simulink model "BESS_GFM_PV_GFL_Stage1_R1_3_PV_POWER_READABLE"  (R2026a)
settings: Solver=ode23t  StopTime=0.9  MaxStep=1e-5
InitFcn:
  | run(fullfile(fileparts(get_param(bdroot,'FileName')),'..','scripts','init_bess_pv_stage1_r1.m'));
undefined symbols (not defined in the file): Control, G, S1, S21
libraries: ee_lib x19, nesl_utility x16, fl_lib x9, simulink x3, sl_discontinuities x1
settings Model: Creator=fakebob2004  LastModifiedBy=fakebob2004
settings SimscapeCC: SimscapeLogType=none

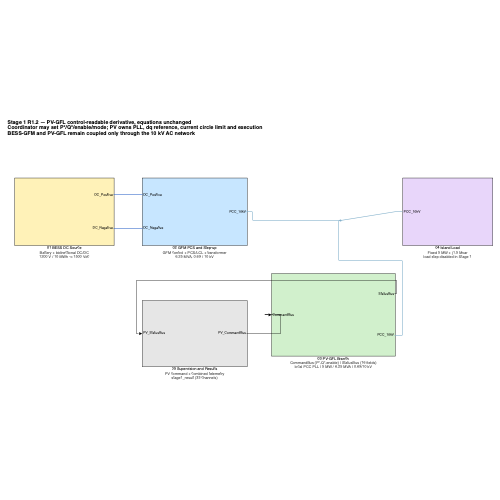
[thumbnail: Simulink's stored preview of the top-level diagram]
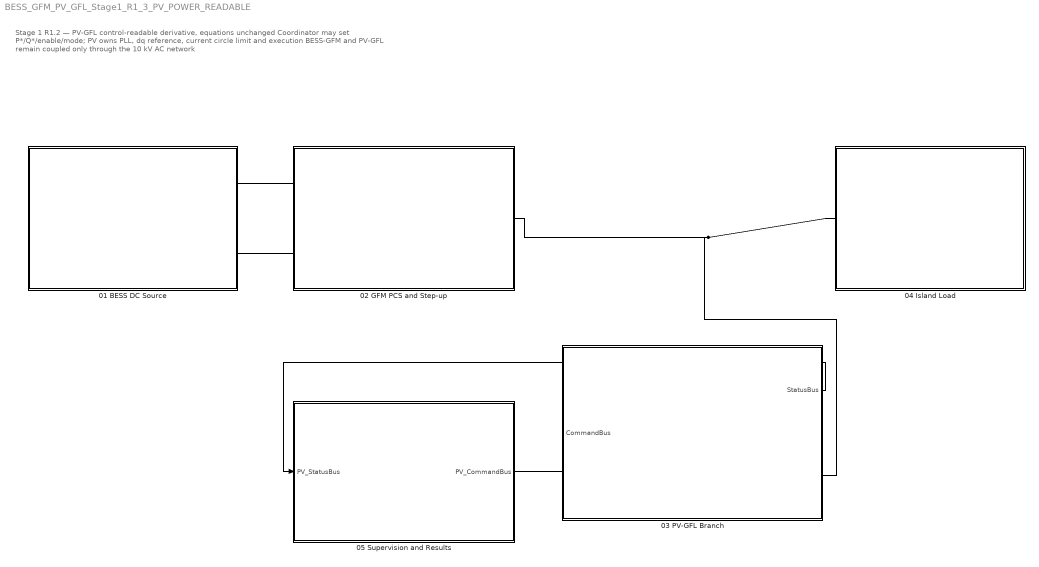
== system BESS_GFM_PV_GFL_Stage1_R1_3_PV_POWER_READABLE ==
  note: Stage 1 R1.2 — PV-GFL control-readable derivative, equations unchanged
      | Coordinator may set P*/Q*/enable/mode; PV owns PLL, dq reference, current circle limit and execution
      | BESS-GFM and PV-GFL remain coupled only through the 10 kV AC network
  01 BESS DC Source : Subsystem
      settings: AttributesFormatString=Battery + bidirectional DC/DC\n1200 V / 10 MWh -> 1500 Vdc
  02 GFM PCS and Step-up : Subsystem
      settings: AttributesFormatString=GFM control + PCS/LCL + transformer\n6.25 MVA, 0.69 / 10 kV
  03 PV-GFL Branch : Subsystem
      settings: AttributesFormatString=|
      | CommandBus {P*,Q*,enable} | StatusBus {16 fields}
      | local PCC PLL | 5 MW / 6.25 MVA | 0.69/10 kV
  04 Island Load : Subsystem
      settings: AttributesFormatString=Fixed 5 MW + j1.5 Mvar\nload step disabled in Stage 1
  05 Supervision and Results : Subsystem
      settings: AttributesFormatString=PV command + combined telemetry\nstage1_result (33 channels)
  wires:
  05 Supervision and Results/1(PV_CommandBus) -> 03 PV-GFL Branch/1(CommandBus)
  03 PV-GFL Branch/1(StatusBus) -> 05 Supervision and Results/1(PV_StatusBus)
  connections:
  01 BESS DC Source/RConn1 -- 02 GFM PCS and Step-up/LConn1
  01 BESS DC Source/RConn2 -- 02 GFM PCS and Step-up/LConn2
  04 Island Load/LConn1 -- 02 GFM PCS and Step-up/RConn1 -- 03 PV-GFL Branch/RConn1

== system BESS_GFM_PV_GFL_Stage1_R1_3_PV_POWER_READABLE/01 BESS DC Source ==
  01 Battery and DC Link : Subsystem
      settings: AttributesFormatString=1200 V / 10 MWh\n1500 V DC link
  02 Bidirectional DC-DC Control : Subsystem
      settings: AttributesFormatString=Vdc PI: 10 Hz\nIbat PI: 300 Hz
  DC_Positive : PMIOPort  Side=Right  ConnectionType=Connection: foundation.electrical.electrical
  DC_Negative : PMIOPort  Port=2  Side=Right  ConnectionType=Connection: foundation.electrical.electrical
  connections:
  02 Bidirectional DC-DC Control/RConn1 -- 01 Battery and DC Link/LConn2
  01 Battery and DC Link/RConn2 -- DC_Negative/RConn1
  DC_Positive/RConn1 -- 01 Battery and DC Link/LConn1

== system BESS_GFM_PV_GFL_Stage1_R1_3_PV_POWER_READABLE/02 GFM PCS and Step-up ==
  03 GFM Control and Limits : Subsystem
      settings: AttributesFormatString=P-f / Q-V / Virtual Z\nAC limit: 1.20 pu
  04 PCS Filter and Transformer : Subsystem
      settings: AttributesFormatString=6.25 MVA PCS + LCL\n0.69 / 10 kV transformer
  DC_Positive : PMIOPort  Side=Left  ConnectionType=Connection: foundation.electrical.electrical
  DC_Negative : PMIOPort  Port=2  Side=Left  ConnectionType=Connection: foundation.electrical.electrical
  PCC_10kV : PMIOPort  Port=3  Side=Right  ConnectionType=Connection: foundation.electrical.three_phase
  connections:
  04 PCS Filter and Transformer/RConn3 -- DC_Negative/RConn1
  04 PCS Filter and Transformer/RConn2 -- PCC_10kV/RConn1
  04 PCS Filter and Transformer/RConn1 -- DC_Positive/RConn1
  03 GFM Control and Limits/RConn1 -- 04 PCS Filter and Transformer/LConn1

== system BESS_GFM_PV_GFL_Stage1_R1_3_PV_POWER_READABLE/03 PV-GFL Branch ==
  CommandBus : Inport
  01 GFL PCS : Subsystem
      settings: AttributesFormatString=|
      | local fast control + average PCS/filter
      | no shared theta, PLL or DC link
  02 Step-up and PCC : Subsystem
      settings: AttributesFormatString=|
      | POWER: 690 V -> 0.69/10 kV -> PCC sensor -> 10 kV
      | MEASUREMENT: local V/I/P/Q -> PCC MeasurementBus
  scope_R21_CurrentCommandBus : GotoTagVisibility  GotoTag=R21_CurrentCommandBus
  scope_R21_PCCMeasurementBus : GotoTagVisibility  GotoTag=R21_PCCMeasurementBus
  scope_R21_PrimaryMeasurementBus : GotoTagVisibility  GotoTag=R21_PrimaryMeasurementBus
  PCC_10kV : PMIOPort  Side=Right  ConnectionType=Connection: foundation.electrical.three_phase
  StatusBus : Outport
  wires:
  01 GFL PCS/1(StatusBus) -> StatusBus/1
  CommandBus/1 -> 01 GFL PCS/1(CommandBus)
  connections:
  01 GFL PCS/RConn1 -- 02 Step-up and PCC/LConn1
  02 Step-up and PCC/RConn1 -- PCC_10kV/RConn1

== system BESS_GFM_PV_GFL_Stage1_R1_3_PV_POWER_READABLE/04 Island Load ==
  Adjusted_Island_Load : ee_lib/Passive/Constant Power Load (Three-Phase)  port_option=ee.enum.threePhasePort.composite  FRated=G.f0_Hz Hz  active_power=G.load.base_P_W W  reactive_power=G.load.base_Q_var V*A  Vline_rms_min=0.70*G.ac.Vll_high_V V  tau=0.01 s  Vline_rms_ini=G.ac.Vll_high_V V  Vang_ini=0 deg  gmin=1e-6 S
  Load_Step_Command : Step  Time=G.load.step_time_s  InitialValue=1  FinalValue=0  SampleTime=0
  Load_Step_to_PS : nesl_utility/Simulink-PS Converter  PhysicalDomain=network_engine_domain  SubClassName=ps_input  LeftPortType=input  RightPortType=output  PseudoPeriodic=off  Frequencies=[]  NoiseDistribution=none  NoiseParameters=[]  Unit=V  AffineConversion=off  FilteringAndDerivatives=zero  SimscapeFilterOrder=1  InputFilterTimeConstant=0.001  UdotUserProvided=0
  One_MW_Step_Load : ee_lib/Passive/Constant Power Load (Three-Phase)  port_option=ee.enum.threePhasePort.composite  FRated=G.f0_Hz Hz  active_power=0 W  reactive_power=0 V*A  Vline_rms_min=0.70*G.ac.Vll_high_V V  tau=0.01 s  Vline_rms_ini=G.ac.Vll_high_V V  Vang_ini=0 deg  gmin=1e-6 S
  Step_Load_Breaker : ee_lib/Switches & Breakers/Circuit Breaker (Three-Phase)  port_option=ee.enum.threePhasePort.composite  control_port_option=ee.enum.controlport.ps  R_closed=0.001 Ohm  G_open=1e-6 1/Ohm  threshold=0.5 V  breaker_behavior=ee.enum.switches.breakerBehavior.zeroCrossingEnable  i_th=1e-8 A
  PCC_10kV : PMIOPort  Side=Left  ConnectionType=Connection: foundation.electrical.three_phase
  tag scope: R8_05_Island_Load_Scenario_p1_signal=global
  wires:
  Load_Step_Command/1 -> Load_Step_to_PS/1, [R8_05_Island_Load_Scenario_p1_signal]  "step_breaker_cmd"
  connections:
  Step_Load_Breaker/RConn1 -- One_MW_Step_Load/LConn1
  PCC_10kV/RConn1 -- Adjusted_Island_Load/LConn1 -- Step_Load_Breaker/LConn2
  Load_Step_to_PS/RConn1 -- Step_Load_Breaker/LConn1

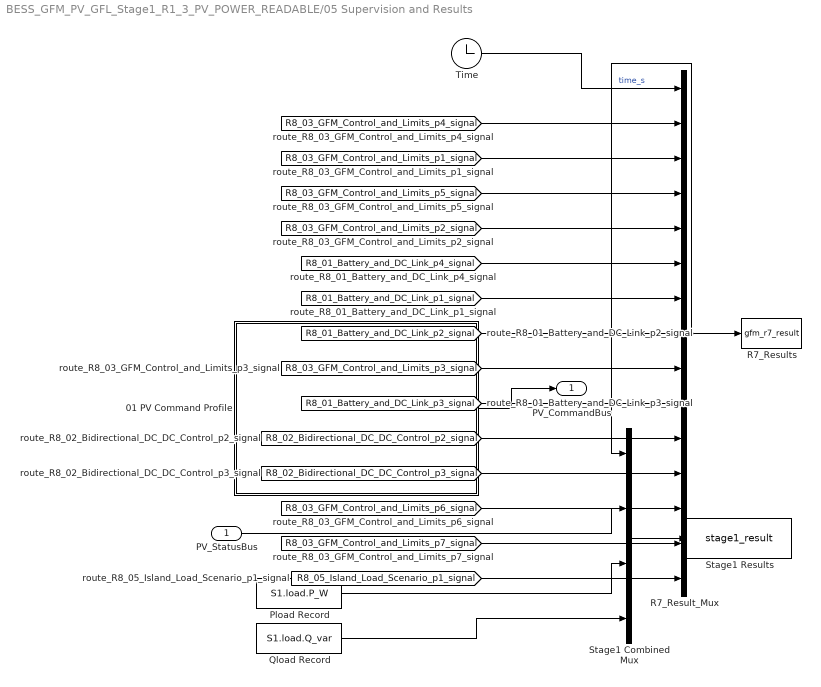
== system BESS_GFM_PV_GFL_Stage1_R1_3_PV_POWER_READABLE/05 Supervision and Results ==
  PV_StatusBus : Inport
  01 PV Command Profile : Subsystem
      settings: AttributesFormatString=|
      | CommandBus = [P*, Q*, enable]
      | commissioning scenario only
  Pload Record : Constant  Value=S1.load.P_W
  Qload Record : Constant  Value=S1.load.Q_var
  R7_Result_Mux : Mux  Inputs=15
  R7_Results : ToWorkspace  VariableName=gfm_r7_result  SampleTime=-1
  Stage1 Combined Mux : Mux
  Stage1 Results : ToWorkspace  VariableName=stage1_result  SampleTime=-1
  Time : Clock
  PV_CommandBus : Outport
  wires:
  [R8_05_Island_Load_Scenario_p1_signal] -> R7_Result_Mux/15
  [R8_03_GFM_Control_and_Limits_p7_signal] -> R7_Result_Mux/14
  R7_Result_Mux/1 -> R7_Results/1, Stage1 Combined Mux/1
  [R8_03_GFM_Control_and_Limits_p6_signal] -> R7_Result_Mux/13
  [R8_02_Bidirectional_DC_DC_Control_p3_signal] -> R7_Result_Mux/12
  [R8_02_Bidirectional_DC_DC_Control_p2_signal] -> R7_Result_Mux/11
  [R8_01_Battery_and_DC_Link_p3_signal] -> R7_Result_Mux/10
  [R8_03_GFM_Control_and_Limits_p3_signal] -> R7_Result_Mux/9
  [R8_01_Battery_and_DC_Link_p2_signal] -> R7_Result_Mux/8
  [R8_01_Battery_and_DC_Link_p1_signal] -> R7_Result_Mux/7
  [R8_01_Battery_and_DC_Link_p4_signal] -> R7_Result_Mux/6
  [R8_03_GFM_Control_and_Limits_p2_signal] -> R7_Result_Mux/5
  Time/1 -> R7_Result_Mux/1  "time_s"
  [R8_03_GFM_Control_and_Limits_p5_signal] -> R7_Result_Mux/4
  [R8_03_GFM_Control_and_Limits_p1_signal] -> R7_Result_Mux/3
  [R8_03_GFM_Control_and_Limits_p4_signal] -> R7_Result_Mux/2
  01 PV Command Profile/1(CommandBus Out) -> PV_CommandBus/1
  PV_StatusBus/1 -> Stage1 Combined Mux/2
  Pload Record/1 -> Stage1 Combined Mux/3
  Qload Record/1 -> Stage1 Combined Mux/4
  Stage1 Combined Mux/1 -> Stage1 Results/1

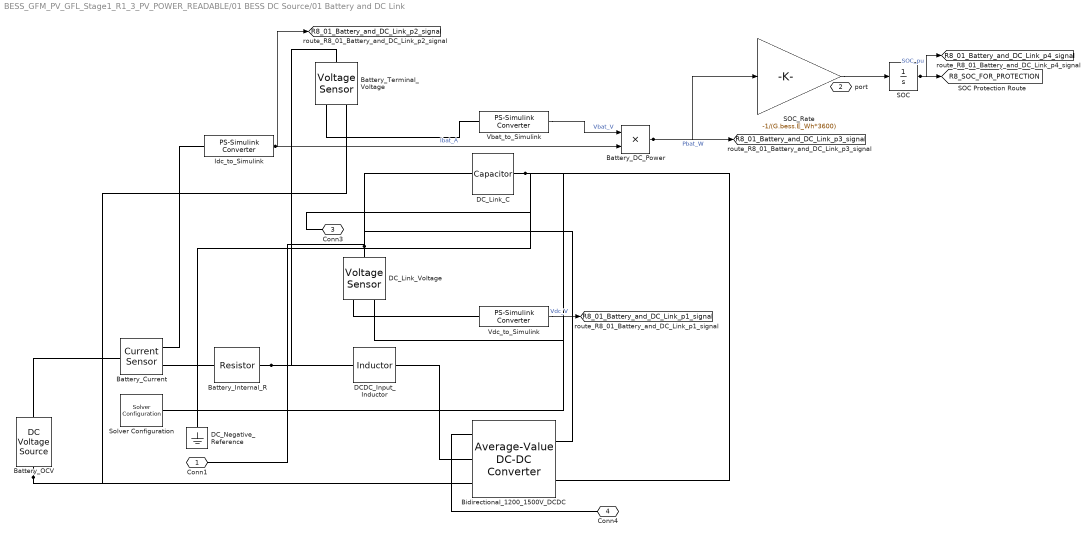
== system BESS_GFM_PV_GFL_Stage1_R1_3_PV_POWER_READABLE/01 BESS DC Source/01 Battery and DC Link ==
  Battery_Current : fl_lib/Electrical/Electrical Sensors/Current Sensor
  Battery_DC_Power : Product
  Battery_Internal_R : fl_lib/Electrical/Electrical Elements/Resistor  R=G.dc.Rbattery_ohm Ohm  i_specify=off  i_priority=None  i=0 A  i_nominal_specify=off  i_nominal_value=1  i_nominal_unit=A  v_specify=off  v_priority=None  v=0 V  v_nominal_specify=off  v_nominal_value=1  v_nominal_unit=V
  Battery_OCV : fl_lib/Electrical/Electrical Sources/DC Voltage Source  v0=G.dc.Vbattery_V V
  Battery_Terminal_Voltage : fl_lib/Electrical/Electrical Sensors/Voltage Sensor
  Bidirectional_1200_1500V_DCDC : ee_lib/Semiconductors & Converters/Converters/Average-Value DC-DC Converter  implementation_option=ee.enum.converters.implementation.behavioral  converter_type=ee.enum.converters.dcdctype.buckboost  control_option=ee.enum.converters.controlinput.dutycycle  efficiency_option=ee.enum.converters.efficiency.constant  efficiency_fixed=G.dc.dcdc_efficiency_pct  i_vec=[0, 2, 5] A  efficiency_vec=[90, 95, 98]  Lf=1e-6 H  Rl=0 Ohm  Cf=1e-7 F  Rc=1e-6 Ohm  iL_specify=off  iL_priority=High  iL=0 A  iL_nominal_specify=off  iL_nominal_value=1  iL_nominal_unit=A  vc_specify=off  vc_priority=High  vc=0 V  vc_nominal_specify=off  vc_nominal_value=1  vc_nominal_unit=V
  DCDC_Input_Inductor : fl_lib/Electrical/Electrical Elements/Inductor  l=G.dcdc.L_H H  r=0 Ohm  g=1e-9 1/Ohm  i_specify=on  i_priority=None  i=G.dcdc.Iref_initial_A A  i_nominal_specify=off  i_nominal_value=1  i_nominal_unit=A  v_specify=off  v_priority=None  v=0 V  v_nominal_specify=off  v_nominal_value=1  v_nominal_unit=V  i_L_specify=off  i_L_priority=High  i_L=0 A  i_L_nominal_specify=off  i_L_nominal_value=1  i_L_nominal_unit=A
  DC_Link_C : fl_lib/Electrical/Electrical Elements/Capacitor  c=G.dc.Cdc_F F  r=1e-6 Ohm  g=0 1/Ohm  i_specify=off  i_priority=None  i=0 A  i_nominal_specify=off  i_nominal_value=1  i_nominal_unit=A  v_specify=off  v_priority=None  v=0 V  v_nominal_specify=off  v_nominal_value=1  v_nominal_unit=V  vc_specify=on  vc_priority=High  vc=G.dc.Vdc_ref_V V  vc_nominal_specify=off  vc_nominal_value=1  vc_nominal_unit=V
  DC_Link_Voltage : fl_lib/Electrical/Electrical Sensors/Voltage Sensor
  DC_Negative_Reference : fl_lib/Electrical/Electrical Elements/Electrical Reference
  Idc_to_Simulink : nesl_utility/PS-Simulink Converter  PhysicalDomain=network_engine_domain  SubClassName=ps_output  LeftPortType=input  RightPortType=output  PseudoPeriodic=off  Frequencies=[]  VectorFormat=inherit  Unit=A  AffineConversion=off
  SOC : Integrator  InitialCondition=G.bess.SOC0  LimitOutput=on  UpperSaturationLimit=G.bess.SOC_max  LowerSaturationLimit=G.bess.SOC_min
  SOC_Rate : Gain  Gain=-1/(G.bess.E_Wh*3600)
  Solver Configuration : nesl_utility/Solver Configuration  PhysicalDomain=network_engine_domain  SubClassName=solver  LeftPortType=input  RightPortType=generic  Tones=[]  Harmonics=[]  SimulateNoise=off  Profile=off  UseLocalSampling=off  EnableSwitchedLinearOptims=on  FrequencyDomain=off  UseCCode=off  RelTol=0.001  AbsTol=0.001  MinStep=1e-09  ToWorkspace=off  RevertToSquareIcSolve=off  NumHomotopyIterations=100  PhasorMode=off  PhasorModeNumHarmonics=1  ConsistencySolver=NEWTON_XTOL_AFTER_FTOL  CanonicalOrdering=CANONICAL  OptimizeIntermediates=OPTIMIZED  IndexReductionMethod=DerivativeReplacement  DoDC=off  ResidualTolerance=1e-09  ConsistencyTolSource=GLOBAL  ConsistencyAbsTol=0.001  ConsistencyRelTol=0.001  ConsistencyTolFactor=0.001  UseLocalSolver=off  LocalSolverChoice=NE_BACKWARD_EULER_ADVANCER  ResolveIndetEquations=on  FunctionEvalNumThread=1  LocalSolverSampleTime=0.001  DoFixedCost=off  MaxNonlinIter=3  MaxModeIter=2  ComputeImpulses=off  ImpulseIterations=2  LinearAlgebra=auto  LinearAlgebraNumThread=0  EquationFormulation=NE_TIME_EF  DelaysMemoryBudget=1024  AutomaticFiltering=on  FilteringTimeConstant=0.001  PartitionStorageMethod=AS_NEEDED  PartitionMemoryBudget=1024  PartitionMethod=ROBUST  MultibodyUseLocalSolver=off  MultibodyLocalSolverChoice=ODE1  MultibodyLocalSolverSampleTime=0.001
  Vbat_to_Simulink : nesl_utility/PS-Simulink Converter  PhysicalDomain=network_engine_domain  SubClassName=ps_output  LeftPortType=input  RightPortType=output  PseudoPeriodic=off  Frequencies=[]  VectorFormat=inherit  Unit=V  AffineConversion=off
  Vdc_to_Simulink : nesl_utility/PS-Simulink Converter  PhysicalDomain=network_engine_domain  SubClassName=ps_output  LeftPortType=input  RightPortType=output  PseudoPeriodic=off  Frequencies=[]  VectorFormat=inherit  Unit=V  AffineConversion=off
  Conn1 : PMIOPort  Side=Left
  port : PMIOPort  Port=2  Side=Right
  Conn3 : PMIOPort  Port=3  Side=Right
  Conn4 : PMIOPort  Port=4  Side=Left
  tag scope: R8_01_Battery_and_DC_Link_p1_signal=global, R8_01_Battery_and_DC_Link_p2_signal=global, R8_01_Battery_and_DC_Link_p3_signal=global, R8_01_Battery_and_DC_Link_p4_signal=global, R8_SOC_FOR_PROTECTION=global
  wires:
  SOC/1 -> [R8_01_Battery_and_DC_Link_p4_signal], [R8_SOC_FOR_PROTECTION]  "SOC_pu"
  Battery_DC_Power/1 -> SOC_Rate/1, [R8_01_Battery_and_DC_Link_p3_signal]  "Pbat_W"
  Vbat_to_Simulink/1 -> Battery_DC_Power/1  "Vbat_V"
  Vdc_to_Simulink/1 -> [R8_01_Battery_and_DC_Link_p1_signal]  "Vdc_V"
  SOC_Rate/1 -> SOC/1
  Idc_to_Simulink/1 -> [R8_01_Battery_and_DC_Link_p2_signal], Battery_DC_Power/2  "Ibat_A"
  connections:
  Conn4/RConn1 -- Bidirectional_1200_1500V_DCDC/LConn1
  DC_Link_Voltage/LConn1 -- Bidirectional_1200_1500V_DCDC/RConn1 -- DC_Link_C/LConn1 -- Conn1/RConn1
  Battery_Terminal_Voltage/RConn1 -- Vbat_to_Simulink/LConn1
  DC_Link_Voltage/RConn1 -- Vdc_to_Simulink/LConn1
  Battery_Internal_R/RConn1 -- DCDC_Input_Inductor/LConn1 -- Battery_Terminal_Voltage/LConn1
  Battery_Current/RConn2 -- Battery_Internal_R/LConn1
  DCDC_Input_Inductor/RConn1 -- Bidirectional_1200_1500V_DCDC/LConn2
  Battery_Current/RConn1 -- Idc_to_Simulink/LConn1
  Battery_OCV/LConn1 -- Battery_Current/LConn1
  DC_Negative_Reference/LConn1 -- DC_Link_C/RConn1 -- Bidirectional_1200_1500V_DCDC/RConn2 -- DC_Link_Voltage/RConn2 -- Conn3/RConn1 -- Solver Configuration/RConn1
  Battery_OCV/RConn1 -- Battery_Terminal_Voltage/RConn2 -- Bidirectional_1200_1500V_DCDC/LConn3

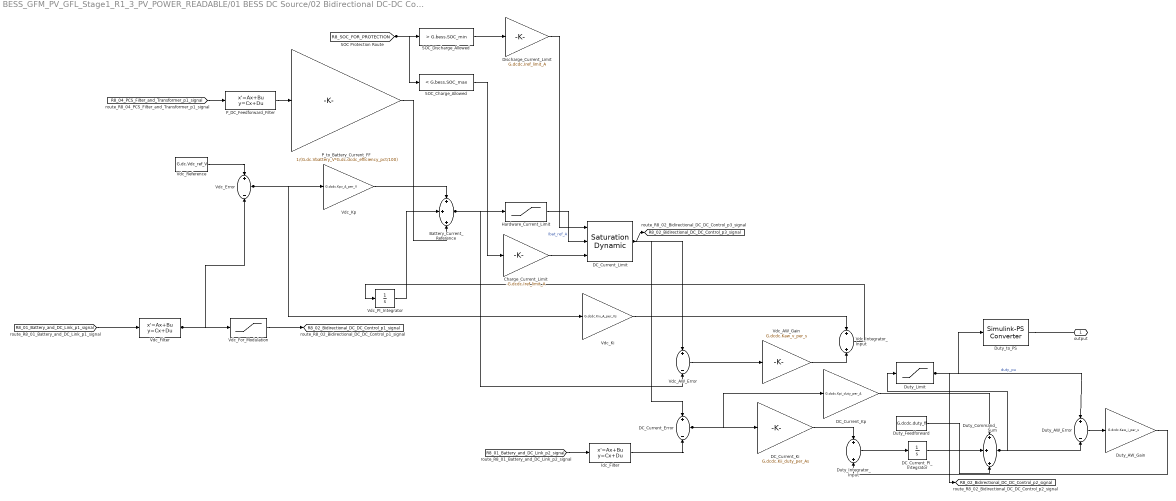
== system BESS_GFM_PV_GFL_Stage1_R1_3_PV_POWER_READABLE/01 BESS DC Source/02 Bidirectional DC-DC Control ==
  Battery_Current_Reference : Sum  Inputs=+++
  Charge_Current_Limit : Gain  Gain=-G.dcdc.Iref_limit_A
  DC_Current_Error : Sum  Inputs=+-
  DC_Current_Ki : Gain  Gain=G.dcdc.Kii_duty_per_As
  DC_Current_Kp : Gain  Gain=G.dcdc.Kpi_duty_per_A
  DC_Current_Limit : sl_discontinuities/Saturation Dynamic  OutMin=[]  OutMax=[]  OutDataTypeStr=Inherit: Same as second input  OutDataType=fixdt(1, 16)  OutScaling=2^-10  DoSatur=off
      settings: LibrarySourceBlock=|
      | simulink/Discontinuities/Saturation
      | Dynamic
  DC_Current_PI_Integrator : Integrator
  Discharge_Current_Limit : Gain  Gain=G.dcdc.Iref_limit_A
  Duty_AW_Error : Sum  Inputs=+-
  Duty_AW_Gain : Gain  Gain=G.dcdc.Kaw_i_per_s
  Duty_Command_Sum : Sum  Inputs=+++
  Duty_Feedforward : Constant  Value=G.dcdc.duty_ff
  Duty_Integrator_Input : Sum
  Duty_Limit : Saturate  UpperLimit=G.dcdc.duty_max  LowerLimit=G.dcdc.duty_min
  Duty_to_PS : nesl_utility/Simulink-PS Converter  PhysicalDomain=network_engine_domain  SubClassName=ps_input  LeftPortType=input  RightPortType=output  PseudoPeriodic=off  Frequencies=[]  NoiseDistribution=none  NoiseParameters=[]  Unit=1  AffineConversion=off  FilteringAndDerivatives=zero  SimscapeFilterOrder=1  InputFilterTimeConstant=0.001  UdotUserProvided=0
  Hardware_Current_Limit : Saturate  UpperLimit=G.dcdc.Iref_limit_A  LowerLimit=-G.dcdc.Iref_limit_A
  Idc_Filter : StateSpace  A=-1/G.dcdc.current_sensor_s  B=1/G.dcdc.current_sensor_s  D=0  InitialCondition=G.dcdc.Iref_initial_A
  P_DC_Feedforward_Filter : StateSpace  A=-1/G.dcdc.power_ff_filter_s  B=1/G.dcdc.power_ff_filter_s  D=0  InitialCondition=G.load.base_P_W
  P_to_Battery_Current_FF : Gain  Gain=1/(G.dc.Vbattery_V*G.dc.dcdc_efficiency_pct/100)
  SOC_Charge_Allowed : simulink/Logic and Bit Operations/Compare To Constant  relop=<  const=G.bess.SOC_max  OutDataTypeStr=boolean
  SOC_Discharge_Allowed : simulink/Logic and Bit Operations/Compare To Constant  relop=>  const=G.bess.SOC_min  OutDataTypeStr=boolean
  Vdc_AW_Error : Sum  Inputs=+-
  Vdc_AW_Gain : Gain  Gain=G.dcdc.Kaw_v_per_s
  Vdc_Error : Sum  Inputs=+-
  Vdc_Filter : StateSpace  A=-1/G.control.Vdc_filter_s  B=1/G.control.Vdc_filter_s  D=0  InitialCondition=G.dc.Vdc_ref_V
  Vdc_For_Modulation : Saturate  UpperLimit=2000  LowerLimit=500
  Vdc_Integrator_Input : Sum
  Vdc_Ki : Gain  Gain=G.dcdc.Kiv_A_per_Vs
  Vdc_Kp : Gain  Gain=G.dcdc.Kpv_A_per_V
  Vdc_PI_Integrator : Integrator
  Vdc_Reference : Constant  Value=G.dc.Vdc_ref_V
  output : PMIOPort  Side=Right
  tag scope: R8_02_Bidirectional_DC_DC_Control_p1_signal=global, R8_02_Bidirectional_DC_DC_Control_p2_signal=global, R8_02_Bidirectional_DC_DC_Control_p3_signal=global
  wires:
  Duty_AW_Gain/1 -> Duty_Integrator_Input/2
  Duty_Limit/1 -> [R8_02_Bidirectional_DC_DC_Control_p2_signal], Duty_AW_Error/1, Duty_to_PS/1  "duty_pu"
  Duty_Integrator_Input/1 -> DC_Current_PI_Integrator/1
  DC_Current_Error/1 -> DC_Current_Ki/1, DC_Current_Kp/1
  Idc_Filter/1 -> DC_Current_Error/2
  Discharge_Current_Limit/1 -> DC_Current_Limit/1
  Vdc_Ki/1 -> Vdc_Integrator_Input/1
  SOC_Charge_Allowed/1 -> Charge_Current_Limit/1
  DC_Current_Limit/1 -> [R8_02_Bidirectional_DC_DC_Control_p3_signal], DC_Current_Error/1, Vdc_AW_Error/1
  [R8_01_Battery_and_DC_Link_p2_signal] -> Idc_Filter/1
  Vdc_AW_Error/1 -> Vdc_AW_Gain/1
  Charge_Current_Limit/1 -> DC_Current_Limit/3
  Hardware_Current_Limit/1 -> DC_Current_Limit/2  "Ibat_ref_A"
  Vdc_Integrator_Input/1 -> Vdc_PI_Integrator/1
  Battery_Current_Reference/1 -> Hardware_Current_Limit/1, Vdc_AW_Error/2
  DC_Current_PI_Integrator/1 -> Duty_Command_Sum/2
  SOC_Discharge_Allowed/1 -> Discharge_Current_Limit/1
  Vdc_PI_Integrator/1 -> Battery_Current_Reference/2
  [R8_04_PCS_Filter_and_Transformer_p1_signal] -> P_DC_Feedforward_Filter/1
  Duty_Feedforward/1 -> Duty_Command_Sum/3
  Vdc_For_Modulation/1 -> [R8_02_Bidirectional_DC_DC_Control_p1_signal]
  [R8_SOC_FOR_PROTECTION] -> SOC_Discharge_Allowed/1, SOC_Charge_Allowed/1
  Vdc_Error/1 -> Vdc_Kp/1, Vdc_Ki/1
  Duty_AW_Error/1 -> Duty_AW_Gain/1
  Vdc_AW_Gain/1 -> Vdc_Integrator_Input/2
  Vdc_Reference/1 -> Vdc_Error/1
  [R8_01_Battery_and_DC_Link_p1_signal] -> Vdc_Filter/1
  DC_Current_Ki/1 -> Duty_Integrator_Input/1
  P_DC_Feedforward_Filter/1 -> P_to_Battery_Current_FF/1
  Vdc_Kp/1 -> Battery_Current_Reference/1
  DC_Current_Kp/1 -> Duty_Command_Sum/1
  P_to_Battery_Current_FF/1 -> Battery_Current_Reference/3
  Duty_Command_Sum/1 -> Duty_AW_Error/2, Duty_Limit/1
  Vdc_Filter/1 -> Vdc_For_Modulation/1, Vdc_Error/2
  connections:
  Duty_to_PS/RConn1 -- output/RConn1

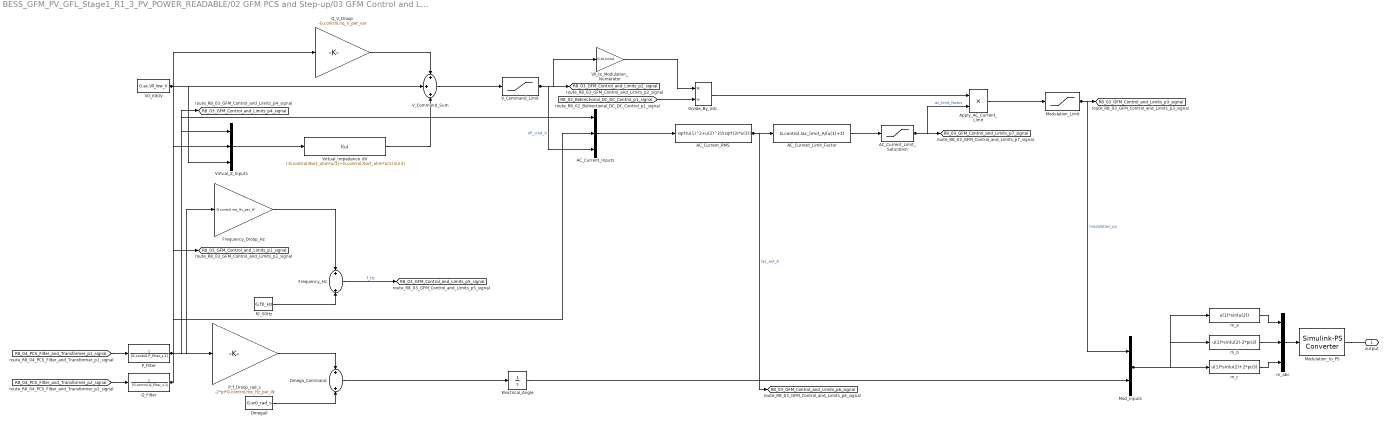
== system BESS_GFM_PV_GFL_Stage1_R1_3_PV_POWER_READABLE/02 GFM PCS and Step-up/03 GFM Control and Limits ==
  AC_Current_Inputs : Mux  Inputs=3
  AC_Current_Limit_Factor : Fcn  Expr=G.control.Iac_limit_A/(u(1)+1)
  AC_Current_Limit_Saturation : Saturate  UpperLimit=1  LowerLimit=0
  AC_Current_RMS : Fcn  Expr=sqrt(u(1)^2+u(2)^2)/(sqrt(3)*u(3))
  Apply_AC_Current_Limit : Product
  Divide_By_Vdc : Product  Inputs=*/
  Electrical_Angle : Integrator  InitialCondition=pi/6
  Frequency_Droop_Hz : Gain  Gain=-G.control.mp_Hz_per_W
  Frequency_Hz : Sum
  Mod_Inputs : Mux  Inputs=2
  Modulation_Limit : Saturate  UpperLimit=G.dc.modulation_max  LowerLimit=0
  Modulation_to_PS : nesl_utility/Simulink-PS Converter  PhysicalDomain=network_engine_domain  SubClassName=ps_input  LeftPortType=input  RightPortType=output  PseudoPeriodic=off  Frequencies=[]  NoiseDistribution=none  NoiseParameters=[]  Unit=1  AffineConversion=off  FilteringAndDerivatives=zero  SimscapeFilterOrder=1  InputFilterTimeConstant=0.001  UdotUserProvided=0
  Omega0 : Constant  Value=G.w0_rad_s
  Omega_Command : Sum
  P_Filter : TransferFcn  Numerator=1  Denominator=[G.control.P_filter_s 1]
  P_f_Droop_rad_s : Gain  Gain=-2*pi*G.control.mp_Hz_per_W
  Q_Filter : TransferFcn  Numerator=1  Denominator=[G.control.Q_filter_s 1]
  Q_V_Droop : Gain  Gain=-G.control.nq_V_per_var
  V0_690V : Constant  Value=G.ac.Vll_low_V
  V_Command_Limit : Saturate  UpperLimit=1.10*G.ac.Vll_low_V  LowerLimit=0.90*G.ac.Vll_low_V
  V_Command_Sum : Sum  Inputs=+++
  Virtual_Impedance_dV : Fcn  Expr=(-G.control.Rvirt_ohm*u(1)+G.control.Xvirt_ohm*u(2))/u(3)
  Virtual_Z_Inputs : Mux  Inputs=3
  Vll_to_Modulation_Numerator : Gain  Gain=G.dc.kmod
  f0_50Hz : Constant  Value=G.f0_Hz
  m_a : Fcn  Expr=u(1)*sin(u(2))
  m_abc : Mux  Inputs=3
  m_b : Fcn  Expr=u(1)*sin(u(2)-2*pi/3)
  m_c : Fcn  Expr=u(1)*sin(u(2)+2*pi/3)
  output : PMIOPort  Side=Right
  tag scope: R8_03_GFM_Control_and_Limits_p1_signal=global, R8_03_GFM_Control_and_Limits_p2_signal=global, R8_03_GFM_Control_and_Limits_p3_signal=global, R8_03_GFM_Control_and_Limits_p4_signal=global, R8_03_GFM_Control_and_Limits_p5_signal=global, R8_03_GFM_Control_and_Limits_p6_signal=global, R8_03_GFM_Control_and_Limits_p7_signal=global
  wires:
  m_abc/1 -> Modulation_to_PS/1
  m_c/1 -> m_abc/3
  m_b/1 -> m_abc/2
  Mod_Inputs/1 -> m_a/1, m_b/1, m_c/1
  m_a/1 -> m_abc/1
  Modulation_Limit/1 -> Mod_Inputs/1, [R8_03_GFM_Control_and_Limits_p3_signal]  "modulation_pu"
  AC_Current_Limit_Saturation/1 -> Apply_AC_Current_Limit/2, [R8_03_GFM_Control_and_Limits_p7_signal]  "ac_limit_factor"
  V_Command_Sum/1 -> V_Command_Limit/1
  Divide_By_Vdc/1 -> Apply_AC_Current_Limit/1
  AC_Current_Inputs/1 -> AC_Current_RMS/1
  [R8_02_Bidirectional_DC_DC_Control_p1_signal] -> Divide_By_Vdc/2
  Vll_to_Modulation_Numerator/1 -> Divide_By_Vdc/1
  Apply_AC_Current_Limit/1 -> Modulation_Limit/1
  V_Command_Limit/1 -> Vll_to_Modulation_Numerator/1, AC_Current_Inputs/3, [R8_03_GFM_Control_and_Limits_p2_signal]  "Vll_cmd_V"
  Virtual_Z_Inputs/1 -> Virtual_Impedance_dV/1
  Frequency_Hz/1 -> [R8_03_GFM_Control_and_Limits_p5_signal]  "f_Hz"
  Virtual_Impedance_dV/1 -> V_Command_Sum/3
  Omega0/1 -> Omega_Command/2
  AC_Current_Limit_Factor/1 -> AC_Current_Limit_Saturation/1
  P_f_Droop_rad_s/1 -> Omega_Command/1
  AC_Current_RMS/1 -> AC_Current_Limit_Factor/1, [R8_03_GFM_Control_and_Limits_p6_signal]  "Iac_est_A"
  Q_V_Droop/1 -> V_Command_Sum/1
  f0_50Hz/1 -> Frequency_Hz/2
  P_Filter/1 -> P_f_Droop_rad_s/1, [R8_03_GFM_Control_and_Limits_p4_signal], AC_Current_Inputs/1, Frequency_Droop_Hz/1, Virtual_Z_Inputs/1
  Frequency_Droop_Hz/1 -> Frequency_Hz/1
  Electrical_Angle/1 -> Mod_Inputs/2
  Omega_Command/1 -> Electrical_Angle/1
  [R8_04_PCS_Filter_and_Transformer_p2_signal] -> Q_Filter/1
  V0_690V/1 -> Virtual_Z_Inputs/3, V_Command_Sum/2
  Q_Filter/1 -> [R8_03_GFM_Control_and_Limits_p1_signal], Virtual_Z_Inputs/2, AC_Current_Inputs/2, Q_V_Droop/1
  [R8_04_PCS_Filter_and_Transformer_p1_signal] -> P_Filter/1
  connections:
  Modulation_to_PS/RConn1 -- output/RConn1

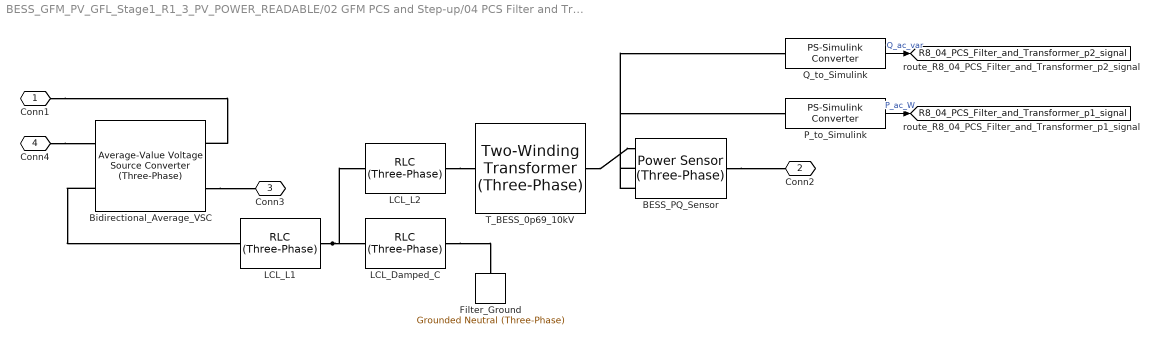
== system BESS_GFM_PV_GFL_Stage1_R1_3_PV_POWER_READABLE/02 GFM PCS and Step-up/04 PCS Filter and Transformer ==
  BESS_PQ_Sensor : ee_lib/Sensors & Transducers/Power Sensor (Three-Phase)  port_option=ee.enum.threePhasePort.composite  load_type=ee.enum.passive.type_balanced.balanced  f0=60 Hz
  Bidirectional_Average_VSC : ee_lib/Semiconductors & Converters/Converters/Average-Value Voltage Source Converter (Three-Phase)  port_option=ee.enum.threePhasePort.composite  enable_block_pulses_input=false  krec=G.dc.Rbattery_ohm/10 Ohm  frequency_option=ee.enum.converters.frequency.variable  input_option=ee.enum.converters.inputOption.ModWave  FRated=G.f0_Hz Hz  losses_parameterization=ee.enum.converters.losses.fixed  Pfixed=1 W  ks=0.01  kc1=1.7 V  kc2=0.01 Ohm  Ploss_vect=[100, 800, 1870, 3250, 4900] W  Irms_vect=[10, 100, 200, 300, 400] A  Vdc_nom=300 V  thermal_mass=30000 J/K  temperature_specify=off  temperature_priority=High  temperature=298.15 K  temperature_nominal_specify=off  temperature_nominal_value=1  temperature_nominal_unit=K
  Filter_Ground : ee_lib/Connectors & References/Grounded Neutral (Three-Phase)  port_option=ee.enum.threePhasePort.composite
  LCL_Damped_C : ee_lib/Passive/RLC Assemblies/RLC (Three-Phase)  port_option=ee.enum.threePhasePort.composite  component_structure=ee.enum.rlc.structure.SeriesRC  R=G.filter.Rd_ohm Ohm  L=1e-3 H  C=G.filter.C_F F  R_parasitic=0 Ohm  G_parasitic=0 1/Ohm  IL_specify=off  IL_priority=High  IL=[0, 0, 0] A  IL_nominal_specify=off  IL_nominal_value=1  IL_nominal_unit=A  VC_specify=off  VC_priority=High  VC=[0, 0, 0] V  VC_nominal_specify=off  VC_nominal_value=1  VC_nominal_unit=V
  LCL_L1 : ee_lib/Passive/RLC Assemblies/RLC (Three-Phase)  port_option=ee.enum.threePhasePort.composite  component_structure=ee.enum.rlc.structure.SeriesRL  R=G.filter.R1_ohm Ohm  L=G.filter.L1_H H  C=1e-6 F  R_parasitic=0 Ohm  G_parasitic=0 1/Ohm  IL_specify=off  IL_priority=High  IL=[0, 0, 0] A  IL_nominal_specify=off  IL_nominal_value=1  IL_nominal_unit=A  VC_specify=off  VC_priority=High  VC=[0, 0, 0] V  VC_nominal_specify=off  VC_nominal_value=1  VC_nominal_unit=V
  LCL_L2 : ee_lib/Passive/RLC Assemblies/RLC (Three-Phase)  port_option=ee.enum.threePhasePort.composite  component_structure=ee.enum.rlc.structure.SeriesRL  R=G.filter.R2_ohm Ohm  L=G.filter.L2_H H  C=1e-6 F  R_parasitic=0 Ohm  G_parasitic=0 1/Ohm  IL_specify=off  IL_priority=High  IL=[0, 0, 0] A  IL_nominal_specify=off  IL_nominal_value=1  IL_nominal_unit=A  VC_specify=off  VC_priority=High  VC=[0, 0, 0] V  VC_nominal_specify=off  VC_nominal_value=1  VC_nominal_unit=V
  P_to_Simulink : nesl_utility/PS-Simulink Converter  PhysicalDomain=network_engine_domain  SubClassName=ps_output  LeftPortType=input  RightPortType=output  PseudoPeriodic=off  Frequencies=[]  VectorFormat=inherit  Unit=W  AffineConversion=off
  Q_to_Simulink : nesl_utility/PS-Simulink Converter  PhysicalDomain=network_engine_domain  SubClassName=ps_output  LeftPortType=input  RightPortType=output  PseudoPeriodic=off  Frequencies=[]  VectorFormat=inherit  Unit=W  AffineConversion=off
  T_BESS_0p69_10kV : ee_lib/Passive/Transformers/Two-Winding Transformer (Three-Phase)  SRated=G.transformer.S_VA A*V  FRated=G.f0_Hz Hz  Winding1Connection=ee.enum.windingconnection.delta1  VRated1=G.ac.Vll_low_V V  Winding2Connection=ee.enum.windingconnection.Yg  VRated2=G.ac.Vll_high_V V  CoreType=ee.enum.coretype.threelimb  pu_Rw1=G.transformer.pu_Rw1  pu_Rw2=G.transformer.pu_Rw2  leakage_reactance_option=ee.enum.transformer_leakage.include  pu_Xl1=G.transformer.pu_Xl1  pu_Xl2=G.transformer.pu_Xl2  magnetizing_resistance_option=ee.enum.transformer_magnetizingResistance.exclude  pu_Rm=500  magnetizing_reactance_option=ee.enum.transformer_magnetizingReactance.exclude  saturation_option=ee.enum.transformer_saturation.exclude  pu_Xm=500  current_data=[0, .002, 1, 2]  magnetic_flux_data=[0, 1.2, 1.5, 1.51]  pu_X0=0.5  i1_specify=off  i1_priority=None  i1=[0, 0, 0] A  i1_nominal_specify=off  i1_nominal_value=1  i1_nominal_unit=A  i2_specify=off  i2_priority=None  i2=[0, 0, 0] A  i2_nominal_specify=off  i2_nominal_value=1  i2_nominal_unit=A  phi_specify=off  phi_priority=None  phi=[0, 0, 0]  phi_nominal_specify=off  phi_nominal_value=1  phi_nominal_unit=1
  Conn1 : PMIOPort  Side=Right  ConnectionType=Connection: foundation.electrical.electrical
  Conn2 : PMIOPort  Port=2  Side=Right  ConnectionType=Connection: foundation.electrical.three_phase
  Conn3 : PMIOPort  Port=3  Side=Right  ConnectionType=Connection: foundation.electrical.electrical
  Conn4 : PMIOPort  Port=4  Side=Left
  tag scope: R8_04_PCS_Filter_and_Transformer_p1_signal=global, R8_04_PCS_Filter_and_Transformer_p2_signal=global
  wires:
  P_to_Simulink/1 -> [R8_04_PCS_Filter_and_Transformer_p1_signal]  "P_ac_W"
  Q_to_Simulink/1 -> [R8_04_PCS_Filter_and_Transformer_p2_signal]  "Q_ac_var"
  connections:
  BESS_PQ_Sensor/RConn1 -- Conn2/RConn1
  BESS_PQ_Sensor/LConn3 -- Q_to_Simulink/LConn1
  LCL_Damped_C/RConn1 -- Filter_Ground/LConn1
  LCL_L2/RConn1 -- T_BESS_0p69_10kV/LConn1
  Bidirectional_Average_VSC/RConn2 -- Conn3/RConn1
  LCL_L1/RConn1 -- LCL_L2/LConn1 -- LCL_Damped_C/LConn1
  T_BESS_0p69_10kV/RConn1 -- BESS_PQ_Sensor/LConn1
  Bidirectional_Average_VSC/LConn2 -- LCL_L1/LConn1
  Conn4/RConn1 -- Bidirectional_Average_VSC/LConn1
  BESS_PQ_Sensor/LConn2 -- P_to_Simulink/LConn1
  Conn1/RConn1 -- Bidirectional_Average_VSC/RConn1

== system BESS_GFM_PV_GFL_Stage1_R1_3_PV_POWER_READABLE/03 PV-GFL Branch/01 GFL PCS ==
  CommandBus : Inport
  01 Secondary Control : Subsystem
      settings: AttributesFormatString=|
      | P/Q command -> dq current -> local execution
      | only compact buses cross this boundary
  02 Primary Converter and Filter : Subsystem
      settings: AttributesFormatString=|
      | average controlled-current PCS
      | interface RL + damped shunt C
  AC_690V : PMIOPort  Side=Right
  StatusBus : Outport
  wires:
  CommandBus/1 -> 01 Secondary Control/1(CommandBus)
  01 Secondary Control/1(StatusBus) -> StatusBus/1
  connections:
  02 Primary Converter and Filter/RConn1 -- AC_690V/RConn1

== system BESS_GFM_PV_GFL_Stage1_R1_3_PV_POWER_READABLE/03 PV-GFL Branch/02 Step-up and PCC ==
  note: THREE-PHASE POWER PATH | 690 V -> transformer -> local PCC sensing -> 10 kV
  note: LOCAL PCC MEASUREMENT ASSEMBLY
  01 PCC Measurement Assembly : Subsystem
      settings: AttributesFormatString=PCC-local V/I/P/Q -> VLL rms + PCC MeasurementBus
  PCC 10kV VI Sensor : ee_lib/Sensors & Transducers/Current and Voltage Sensor (Three-Phase)  port_option=ee.enum.threePhasePort.composite  vMeasurementType=ee.enum.vmeasurement.ll  outputUnit=ee.enum.unit.si  SRated=100e6 A*V  VRated=24e3 V  I_specify=off  I_priority=None  I=[0, 0, 0] A  I_nominal_specify=off  I_nominal_value=1  I_nominal_unit=A  V_specify=off  V_priority=None  V=[0, 0, 0] V  V_nominal_specify=off  V_nominal_value=1  V_nominal_unit=V
  PV PCC Power Sensor : ee_lib/Sensors & Transducers/Power Sensor (Three-Phase)  port_option=ee.enum.threePhasePort.composite  load_type=ee.enum.passive.type_balanced.balanced  f0=60 Hz
  T_PV_0p69_10kV : ee_lib/Passive/Transformers/Two-Winding Transformer (Three-Phase)  SRated=S1.transformer.S_VA A*V  FRated=S1.base.f_Hz Hz  Winding1Connection=ee.enum.windingconnection.Yg  VRated1=S1.pv.Vll_low_V V  Winding2Connection=ee.enum.windingconnection.Yg  VRated2=S1.pv.Vll_high_V V  CoreType=ee.enum.coretype.threelimb  pu_Rw1=S1.transformer.R_pu/2  pu_Rw2=S1.transformer.R_pu/2  leakage_reactance_option=ee.enum.transformer_leakage.exclude  pu_Xl1=0.05  pu_Xl2=0.05  magnetizing_resistance_option=ee.enum.transformer_magnetizingResistance.exclude  pu_Rm=500  magnetizing_reactance_option=ee.enum.transformer_magnetizingReactance.exclude  saturation_option=ee.enum.transformer_saturation.exclude  pu_Xm=500  current_data=[0, .002, 1, 2]  magnetic_flux_data=[0, 1.2, 1.5, 1.51]  pu_X0=0.5  i1_specify=off  i1_priority=None  i1=[0, 0, 0] A  i1_nominal_specify=off  i1_nominal_value=1  i1_nominal_unit=A  i2_specify=off  i2_priority=None  i2=[0, 0, 0] A  i2_nominal_specify=off  i2_nominal_value=1  i2_nominal_unit=A  phi_specify=off  phi_priority=None  phi=[0, 0, 0]  phi_nominal_specify=off  phi_nominal_value=1  phi_nominal_unit=1
  PCC_10kV : PMIOPort  Side=Right
  AC_690V : PMIOPort  Port=2  Side=Left
  tag scope: R21_PCCMeasurementBus=scoped
  wires:
  01 PCC Measurement Assembly/1(Out1) -> [R21_PCCMeasurementBus]
  connections:
  PV PCC Power Sensor/RConn1 -- PCC_10kV/RConn1
  AC_690V/RConn1 -- T_PV_0p69_10kV/LConn1
  PCC 10kV VI Sensor/RConn3 -- PV PCC Power Sensor/LConn1
  T_PV_0p69_10kV/RConn1 -- PCC 10kV VI Sensor/LConn1
  PCC 10kV VI Sensor/RConn1 -- 01 PCC Measurement Assembly/LConn1
  PV PCC Power Sensor/LConn2 -- 01 PCC Measurement Assembly/LConn2
  PV PCC Power Sensor/LConn3 -- 01 PCC Measurement Assembly/LConn3
  PCC 10kV VI Sensor/RConn2 -- 01 PCC Measurement Assembly/LConn4

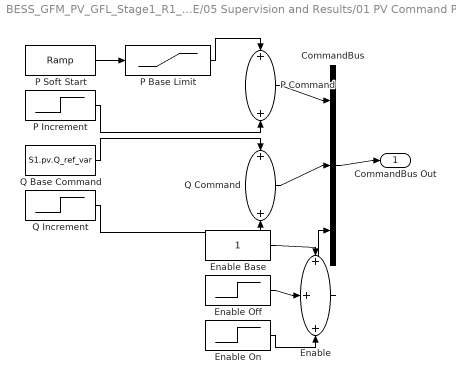
== system BESS_GFM_PV_GFL_Stage1_R1_3_PV_POWER_READABLE/05 Supervision and Results/01 PV Command Profile ==
  CommandBus : Mux  Inputs=3
  Enable : Sum  Inputs=+++
  Enable Base : Constant
  Enable Off : Step  Time=10  FinalValue=0  SampleTime=0
  Enable On : Step  Time=11  FinalValue=0  SampleTime=0
  P Base Limit : Saturate  UpperLimit=S1.pv.P_initial_W  LowerLimit=0
  P Command : Sum
  P Increment : Step  Time=S1.pv.P_step_time_s  FinalValue=S1.pv.P_final_W-S1.pv.P_initial_W  SampleTime=0
  P Soft Start : simulink/Sources/Ramp  slope=S1.pv.P_ramp_W_per_s  start=0  InitialOutput=0
  Q Base Command : Constant  Value=S1.pv.Q_ref_var
  Q Command : Sum
  Q Increment : Step  Time=S1.pv.P_step_time_s  FinalValue=0  SampleTime=0
  CommandBus Out : Outport
  wires:
  Enable/1 -> CommandBus/3
  Enable On/1 -> Enable/3
  Enable Off/1 -> Enable/2
  Enable Base/1 -> Enable/1
  CommandBus/1 -> CommandBus Out/1
  Q Command/1 -> CommandBus/2
  P Command/1 -> CommandBus/1
  Q Increment/1 -> Q Command/2
  Q Base Command/1 -> Q Command/1
  P Increment/1 -> P Command/2
  P Base Limit/1 -> P Command/1
  P Soft Start/1 -> P Base Limit/1

== system BESS_GFM_PV_GFL_Stage1_R1_3_PV_POWER_READABLE/03 PV-GFL Branch/01 GFL PCS/01 Secondary Control ==
  CommandBus : Inport
  01 Local SRF-PLL : Subsystem
      settings: AttributesFormatString=|
      | PV-local 10 kV PCC voltage only
      | wrapped phase-error PI | 45-55 Hz
  02 Current Command Generation : Subsystem
      settings: AttributesFormatString=|
      | P/Q -> dq | enable gate | circle limit
      | 150 Hz tracking -> abc current command
  03 Status Assembly : Subsystem
      settings: AttributesFormatString=|
      | ordered 16-field status vector
      | measurement + command + PLL + limits
  StatusBus : Outport
  wires:
  01 Local SRF-PLL/1(theta) -> 03 Status Assembly/5(In5), 02 Current Command Generation/1(In1)
  CommandBus/1 -> 02 Current Command Generation/2(In2)
  01 Local SRF-PLL/2(Out2) -> 03 Status Assembly/1(In1)
  01 Local SRF-PLL/3(Out3) -> 03 Status Assembly/2(In2)
  01 Local SRF-PLL/4(omega) -> 03 Status Assembly/3(In3)
  01 Local SRF-PLL/5(phase error) -> 03 Status Assembly/4(In4)
  01 Local SRF-PLL/6(Out6) -> 03 Status Assembly/6(In6)
  03 Status Assembly/1(Out1) -> StatusBus/1
  02 Current Command Generation/1(StatusTelemetryBus) -> 03 Status Assembly/7(CurrentGen Status Bus)

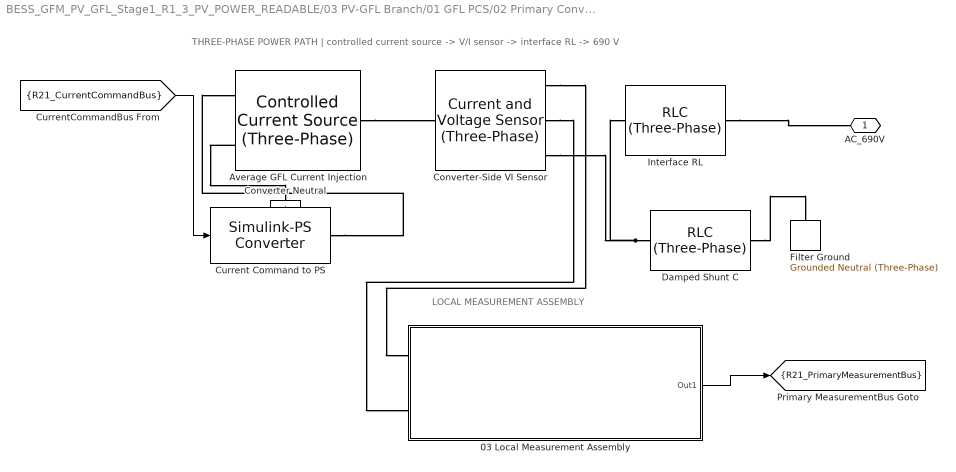
== system BESS_GFM_PV_GFL_Stage1_R1_3_PV_POWER_READABLE/03 PV-GFL Branch/01 GFL PCS/02 Primary Converter and Filter ==
  note: THREE-PHASE POWER PATH | controlled current source -> V/I sensor -> interface RL -> 690 V
  note: LOCAL MEASUREMENT ASSEMBLY
  03 Local Measurement Assembly : Subsystem
      settings: AttributesFormatString=converter-side V/I -> magnitude + Primary MeasurementBus
  Average GFL Current Injection : ee_lib/Sources/Controlled Current Source (Three-Phase)  port_option=ee.enum.threePhasePort.composite  input_option=ee.enum.inputType.instantaneous  FRated=S1.base.f_Hz Hz  G_parasitic=1e-6 1/Ohm
  Converter Neutral : fl_lib/Electrical/Electrical Elements/Electrical Reference
  Converter-Side VI Sensor : ee_lib/Sensors & Transducers/Current and Voltage Sensor (Three-Phase)  port_option=ee.enum.threePhasePort.composite  vMeasurementType=ee.enum.vmeasurement.ll  outputUnit=ee.enum.unit.si  SRated=100e6 A*V  VRated=24e3 V  I_specify=off  I_priority=None  I=[0, 0, 0] A  I_nominal_specify=off  I_nominal_value=1  I_nominal_unit=A  V_specify=off  V_priority=None  V=[0, 0, 0] V  V_nominal_specify=off  V_nominal_value=1  V_nominal_unit=V
  Current Command to PS : nesl_utility/Simulink-PS Converter  PhysicalDomain=network_engine_domain  SubClassName=ps_input  LeftPortType=input  RightPortType=output  PseudoPeriodic=off  Frequencies=[]  NoiseDistribution=none  NoiseParameters=[]  Unit=A  AffineConversion=off  FilteringAndDerivatives=zero  SimscapeFilterOrder=1  InputFilterTimeConstant=0.001  UdotUserProvided=0
  Damped Shunt C : ee_lib/Passive/RLC Assemblies/RLC (Three-Phase)  port_option=ee.enum.threePhasePort.composite  component_structure=ee.enum.rlc.structure.SeriesRC  R=S1.filter.Rd_ohm Ohm  L=1e-3 H  C=S1.filter.C_F F  R_parasitic=0 Ohm  G_parasitic=0 1/Ohm  IL_specify=off  IL_priority=High  IL=[0, 0, 0] A  IL_nominal_specify=off  IL_nominal_value=1  IL_nominal_unit=A  VC_specify=off  VC_priority=High  VC=[0, 0, 0] V  VC_nominal_specify=off  VC_nominal_value=1  VC_nominal_unit=V
  Filter Ground : ee_lib/Connectors & References/Grounded Neutral (Three-Phase)  port_option=ee.enum.threePhasePort.composite
  Interface RL : ee_lib/Passive/RLC Assemblies/RLC (Three-Phase)  port_option=ee.enum.threePhasePort.composite  component_structure=ee.enum.rlc.structure.R  R=S1.filter.R1_ohm+S1.filter.R2_ohm Ohm  L=1e-3 H  C=1e-6 F  R_parasitic=0 Ohm  G_parasitic=0 1/Ohm  IL_specify=off  IL_priority=High  IL=[0, 0, 0] A  IL_nominal_specify=off  IL_nominal_value=1  IL_nominal_unit=A  VC_specify=off  VC_priority=High  VC=[0, 0, 0] V  VC_nominal_specify=off  VC_nominal_value=1  VC_nominal_unit=V
  AC_690V : PMIOPort  Side=Right
  tag scope: R21_PrimaryMeasurementBus=scoped
  wires:
  [R21_CurrentCommandBus] -> Current Command to PS/1
  03 Local Measurement Assembly/1(Out1) -> [R21_PrimaryMeasurementBus]
  connections:
  Damped Shunt C/LConn1 -- Converter-Side VI Sensor/RConn3 -- Interface RL/LConn1
  Current Command to PS/RConn1 -- Average GFL Current Injection/LConn1
  Average GFL Current Injection/LConn2 -- Converter Neutral/LConn1
  Interface RL/RConn1 -- AC_690V/RConn1
  Damped Shunt C/RConn1 -- Filter Ground/LConn1
  Average GFL Current Injection/RConn1 -- Converter-Side VI Sensor/LConn1
  Converter-Side VI Sensor/RConn1 -- 03 Local Measurement Assembly/LConn1
  Converter-Side VI Sensor/RConn2 -- 03 Local Measurement Assembly/LConn2

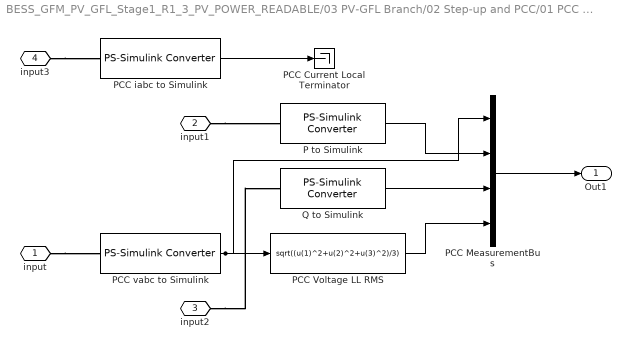
== system BESS_GFM_PV_GFL_Stage1_R1_3_PV_POWER_READABLE/03 PV-GFL Branch/02 Step-up and PCC/01 PCC Measurement Assembly ==
  P to Simulink : nesl_utility/PS-Simulink Converter  PhysicalDomain=network_engine_domain  SubClassName=ps_output  LeftPortType=input  RightPortType=output  PseudoPeriodic=off  Frequencies=[]  VectorFormat=inherit  Unit=W  AffineConversion=off
  PCC Current Local Terminator : Terminator
  PCC MeasurementBus : Mux
  PCC Voltage LL RMS : Fcn  Expr=sqrt((u(1)^2+u(2)^2+u(3)^2)/3)
  PCC iabc to Simulink : nesl_utility/PS-Simulink Converter  PhysicalDomain=network_engine_domain  SubClassName=ps_output  LeftPortType=input  RightPortType=output  PseudoPeriodic=off  Frequencies=[]  VectorFormat=inherit  Unit=A  AffineConversion=off
  PCC vabc to Simulink : nesl_utility/PS-Simulink Converter  PhysicalDomain=network_engine_domain  SubClassName=ps_output  LeftPortType=input  RightPortType=output  PseudoPeriodic=off  Frequencies=[]  VectorFormat=inherit  Unit=V  AffineConversion=off
  Q to Simulink : nesl_utility/PS-Simulink Converter  PhysicalDomain=network_engine_domain  SubClassName=ps_output  LeftPortType=input  RightPortType=output  PseudoPeriodic=off  Frequencies=[]  VectorFormat=inherit  Unit=W  AffineConversion=off
  input : PMIOPort  Side=Left
  input1 : PMIOPort  Port=2  Side=Left
  input2 : PMIOPort  Port=3  Side=Left
  input3 : PMIOPort  Port=4  Side=Left
  Out1 : Outport
  wires:
  PCC MeasurementBus/1 -> Out1/1
  PCC Voltage LL RMS/1 -> PCC MeasurementBus/4
  P to Simulink/1 -> PCC MeasurementBus/2
  PCC vabc to Simulink/1 -> PCC Voltage LL RMS/1, PCC MeasurementBus/1
  Q to Simulink/1 -> PCC MeasurementBus/3
  PCC iabc to Simulink/1 -> PCC Current Local Terminator/1
  connections:
  input2/RConn1 -- Q to Simulink/LConn1
  input/RConn1 -- PCC vabc to Simulink/LConn1
  input1/RConn1 -- P to Simulink/LConn1
  input3/RConn1 -- PCC iabc to Simulink/LConn1

== system BESS_GFM_PV_GFL_Stage1_R1_3_PV_POWER_READABLE/03 PV-GFL Branch/01 GFL PCS/01 Secondary Control/01 Local SRF-PLL ==
  PCC Measurement Selector : Demux  Outputs=[3 1 1 1]
  SRF-PLL Core : Subsystem
      settings: AttributesFormatString=|
      | local abc voltage only
      | wrapped phase-error PI
  theta : Outport
  Out2 : Outport  Port=2
  Out3 : Outport  Port=3
  omega : Outport  Port=4
  phase error : Outport  Port=5
  Out6 : Outport  Port=6
  wires:
  SRF-PLL Core/3(phase error) -> phase error/1
  SRF-PLL Core/1(theta) -> theta/1
  PCC Measurement Selector/4 -> Out6/1
  PCC Measurement Selector/3 -> Out3/1
  PCC Measurement Selector/2 -> Out2/1
  PCC Measurement Selector/1 -> SRF-PLL Core/1(Vabc)
  SRF-PLL Core/2(omega) -> omega/1
  [R21_PCCMeasurementBus] -> PCC Measurement Selector/1

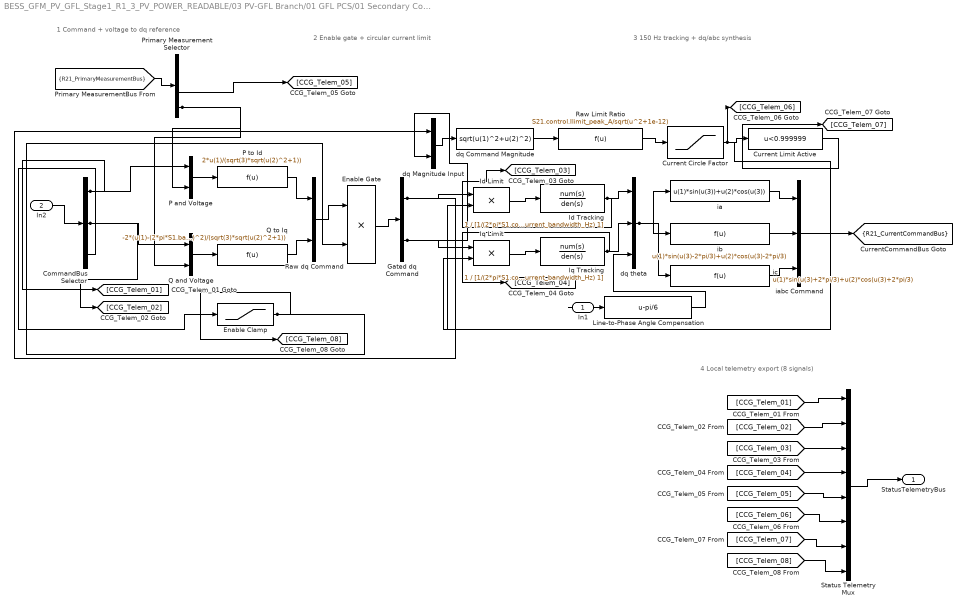
== system BESS_GFM_PV_GFL_Stage1_R1_3_PV_POWER_READABLE/03 PV-GFL Branch/01 GFL PCS/01 Secondary Control/02 Current Command Generation ==
  note: 1 Command + voltage to dq reference
  note: 2 Enable gate + circular current limit
  note: 3 150 Hz tracking + dq/abc synthesis
  note: 4 Local telemetry export (8 signals)
  In1 : Inport
  In2 : Inport  Port=2
  CommandBus Selector : Demux  Outputs=3
  Current Circle Factor : Saturate  UpperLimit=1  LowerLimit=0
  Current Limit Active : Fcn  Expr=u<0.999999
  Enable Clamp : Saturate  UpperLimit=1  LowerLimit=0
  Enable Gate : Product  Inputs=**
  Gated dq Command : Demux  Outputs=2
  Id Limit : Product  Inputs=**
  Id Tracking : TransferFcn  Numerator=1  Denominator=[1/(2*pi*S1.control.current_bandwidth_Hz) 1]
  Iq Limit : Product  Inputs=**
  Iq Tracking : TransferFcn  Numerator=1  Denominator=[1/(2*pi*S1.control.current_bandwidth_Hz) 1]
  Line-to-Phase Angle Compensation : Fcn  Expr=u-pi/6
  P and Voltage : Mux  Inputs=2
  P to Id : Fcn  Expr=2*u(1)/(sqrt(3)*sqrt(u(2)^2+1))
  Primary Measurement Selector : Demux  Outputs=[3 3 1 1]
  Q and Voltage : Mux  Inputs=2
  Q to Iq : Fcn  Expr=-2*(u(1)-(2*pi*S1.base.f_Hz*S1.filter.C_F/2)*u(2)^2)/(sqrt(3)*sqrt(u(2)^2+1))
  Raw Limit Ratio : Fcn  Expr=S21.control.Ilimit_peak_A/sqrt(u^2+1e-12)
  Raw dq Command : Mux  Inputs=2
  Status Telemetry Mux : Mux  Inputs=8
  dq Command Magnitude : Fcn  Expr=sqrt(u(1)^2+u(2)^2)
  dq Magnitude Input : Mux  Inputs=2
  dq theta : Mux  Inputs=3
  ia : Fcn  Expr=u(1)*sin(u(3))+u(2)*cos(u(3))
  iabc Command : Mux  Inputs=3
  ib : Fcn  Expr=u(1)*sin(u(3)-2*pi/3)+u(2)*cos(u(3)-2*pi/3)
  ic : Fcn  Expr=u(1)*sin(u(3)+2*pi/3)+u(2)*cos(u(3)+2*pi/3)
  StatusTelemetryBus : Outport
  tag scope: R21_CurrentCommandBus=scoped
  wires:
  Primary Measurement Selector/3 -> [CCG_Telem_05]
  ia/1 -> iabc Command/1
  Raw Limit Ratio/1 -> Current Circle Factor/1
  In1/1 -> Line-to-Phase Angle Compensation/1
  In2/1 -> CommandBus Selector/1
  Raw dq Command/1 -> Enable Gate/1
  Id Limit/1 -> Id Tracking/1
  Gated dq Command/2 -> Iq Limit/1, dq Magnitude Input/2
  ic/1 -> iabc Command/3
  [R21_PrimaryMeasurementBus] -> Primary Measurement Selector/1
  CommandBus Selector/3 -> Enable Clamp/1
  P and Voltage/1 -> P to Id/1
  Current Limit Active/1 -> [CCG_Telem_07]
  Iq Tracking/1 -> dq theta/2, [CCG_Telem_04]
  Line-to-Phase Angle Compensation/1 -> dq theta/3
  Primary Measurement Selector/4 -> Q and Voltage/2, P and Voltage/2
  Id Tracking/1 -> [CCG_Telem_03], dq theta/1
  dq theta/1 -> ic/1, ib/1, ia/1
  Enable Clamp/1 -> Enable Gate/2, [CCG_Telem_08]
  ib/1 -> iabc Command/2
  P to Id/1 -> Raw dq Command/1
  Q and Voltage/1 -> Q to Iq/1
  dq Magnitude Input/1 -> dq Command Magnitude/1
  CommandBus Selector/1 -> P and Voltage/1, [CCG_Telem_01]
  Enable Gate/1 -> Gated dq Command/1
  Iq Limit/1 -> Iq Tracking/1
  Current Circle Factor/1 -> Iq Limit/2, Id Limit/2, [CCG_Telem_06], Current Limit Active/1
  Q to Iq/1 -> Raw dq Command/2
  dq Command Magnitude/1 -> Raw Limit Ratio/1
  CommandBus Selector/2 -> Q and Voltage/1, [CCG_Telem_02]
  iabc Command/1 -> [R21_CurrentCommandBus]
  Gated dq Command/1 -> Id Limit/1, dq Magnitude Input/1
  [CCG_Telem_01] -> Status Telemetry Mux/1
  [CCG_Telem_02] -> Status Telemetry Mux/2
  [CCG_Telem_03] -> Status Telemetry Mux/3
  [CCG_Telem_04] -> Status Telemetry Mux/4
  [CCG_Telem_05] -> Status Telemetry Mux/5
  [CCG_Telem_06] -> Status Telemetry Mux/6
  [CCG_Telem_07] -> Status Telemetry Mux/7
  [CCG_Telem_08] -> Status Telemetry Mux/8
  Status Telemetry Mux/1 -> StatusTelemetryBus/1

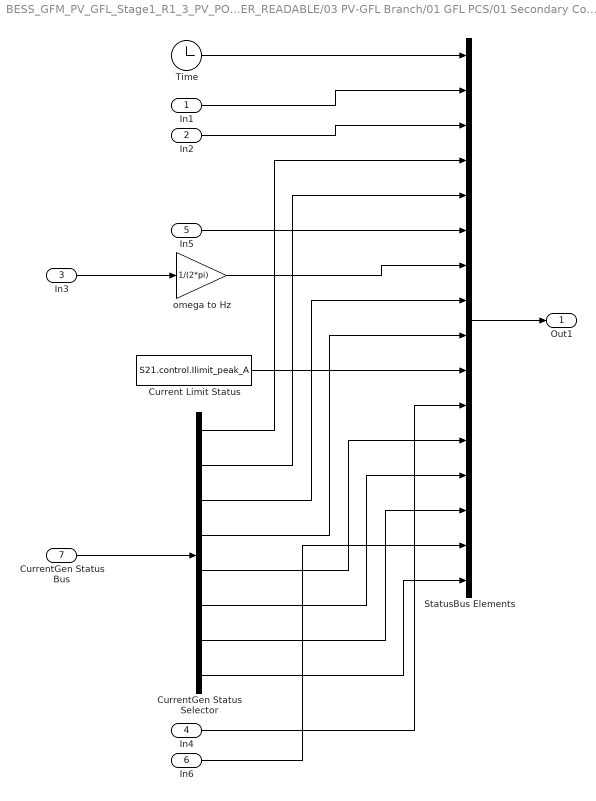
== system BESS_GFM_PV_GFL_Stage1_R1_3_PV_POWER_READABLE/03 PV-GFL Branch/01 GFL PCS/01 Secondary Control/03 Status Assembly ==
  In1 : Inport
  In2 : Inport  Port=2
  In3 : Inport  Port=3
  In4 : Inport  Port=4
  In5 : Inport  Port=5
  In6 : Inport  Port=6
  CurrentGen Status Bus : Inport  Port=7
  Current Limit Status : Constant  Value=S21.control.Ilimit_peak_A
  CurrentGen Status Selector : Demux  Outputs=8
  StatusBus Elements : Mux  Inputs=16
  Time : Clock
  omega to Hz : Gain  Gain=1/(2*pi)
  Out1 : Outport
  wires:
  StatusBus Elements/1 -> Out1/1
  In6/1 -> StatusBus Elements/15
  CurrentGen Status Selector/8 -> StatusBus Elements/16
  CurrentGen Status Selector/7 -> StatusBus Elements/14
  CurrentGen Status Selector/6 -> StatusBus Elements/13
  CurrentGen Status Selector/5 -> StatusBus Elements/12
  CurrentGen Status Selector/4 -> StatusBus Elements/9
  Current Limit Status/1 -> StatusBus Elements/10
  CurrentGen Status Selector/2 -> StatusBus Elements/5
  omega to Hz/1 -> StatusBus Elements/7
  CurrentGen Status Selector/1 -> StatusBus Elements/4
  In5/1 -> StatusBus Elements/6
  In2/1 -> StatusBus Elements/3
  In1/1 -> StatusBus Elements/2
  In4/1 -> StatusBus Elements/11
  CurrentGen Status Bus/1 -> CurrentGen Status Selector/1
  Time/1 -> StatusBus Elements/1
  CurrentGen Status Selector/3 -> StatusBus Elements/8
  In3/1 -> omega to Hz/1

== system BESS_GFM_PV_GFL_Stage1_R1_3_PV_POWER_READABLE/03 PV-GFL Branch/01 GFL PCS/02 Primary Converter and Filter/03 Local Measurement Assembly ==
  Actual Current Magnitude : Fcn  Expr=sqrt((2/3)*(u(1)^2+u(2)^2+u(3)^2))
  Line Voltage Peak Magnitude : Fcn  Expr=sqrt((2/3)*(u(1)^2+u(2)^2+u(3)^2))
  Local Voltage Record : ToWorkspace  VariableName=gfl_r2_vabc  SampleTime=-1
  Primary MeasurementBus : Mux
  iabc to Simulink : nesl_utility/PS-Simulink Converter  PhysicalDomain=network_engine_domain  SubClassName=ps_output  LeftPortType=input  RightPortType=output  PseudoPeriodic=off  Frequencies=[]  VectorFormat=inherit  Unit=A  AffineConversion=off
  vabc to Simulink : nesl_utility/PS-Simulink Converter  PhysicalDomain=network_engine_domain  SubClassName=ps_output  LeftPortType=input  RightPortType=output  PseudoPeriodic=off  Frequencies=[]  VectorFormat=inherit  Unit=V  AffineConversion=off
  input : PMIOPort  Side=Left
  input1 : PMIOPort  Port=2  Side=Left
  Out1 : Outport
  wires:
  Primary MeasurementBus/1 -> Out1/1
  Actual Current Magnitude/1 -> Primary MeasurementBus/3
  iabc to Simulink/1 -> Actual Current Magnitude/1, Primary MeasurementBus/2
  Line Voltage Peak Magnitude/1 -> Primary MeasurementBus/4
  vabc to Simulink/1 -> Local Voltage Record/1, Line Voltage Peak Magnitude/1, Primary MeasurementBus/1
  connections:
  input1/RConn1 -- iabc to Simulink/LConn1
  input/RConn1 -- vabc to Simulink/LConn1

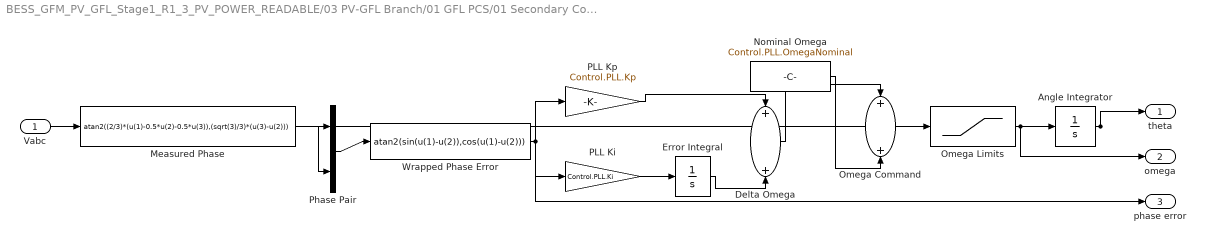
== system BESS_GFM_PV_GFL_Stage1_R1_3_PV_POWER_READABLE/03 PV-GFL Branch/01 GFL PCS/01 Secondary Control/01 Local SRF-PLL/SRF-PLL Core ==
  Vabc : Inport
  Angle Integrator : Integrator  InitialCondition=Control.PLL.Theta0
  Delta Omega : Sum
  Error Integral : Integrator
  Measured Phase : Fcn  Expr=atan2((2/3)*(u(1)-0.5*u(2)-0.5*u(3)),(sqrt(3)/3)*(u(3)-u(2)))
  Nominal Omega : Constant  Value=Control.PLL.OmegaNominal
  Omega Command : Sum
  Omega Limits : Saturate  UpperLimit=Control.PLL.OmegaMax  LowerLimit=Control.PLL.OmegaMin
  PLL Ki : Gain  Gain=Control.PLL.Ki
  PLL Kp : Gain  Gain=Control.PLL.Kp
  Phase Pair : Mux  Inputs=2
  Wrapped Phase Error : Fcn  Expr=atan2(sin(u(1)-u(2)),cos(u(1)-u(2)))
  theta : Outport
  omega : Outport  Port=2
  phase error : Outport  Port=3
  wires:
  Omega Limits/1 -> omega/1, Angle Integrator/1
  Omega Command/1 -> Omega Limits/1
  Nominal Omega/1 -> Omega Command/2
  Delta Omega/1 -> Omega Command/1
  Error Integral/1 -> Delta Omega/2
  PLL Kp/1 -> Delta Omega/1
  PLL Ki/1 -> Error Integral/1
  Wrapped Phase Error/1 -> phase error/1, PLL Ki/1, PLL Kp/1
  Phase Pair/1 -> Wrapped Phase Error/1
  Angle Integrator/1 -> theta/1, Phase Pair/2
  Measured Phase/1 -> Phase Pair/1
  Vabc/1 -> Measured Phase/1
